simulink model "commoteur"  (Simulink 7.0)
settings: Solver=FixedStepDiscrete  StartTime=0.0  StopTime=300  FixedStep=0.0001  RelTol=1e-3
libraries: dsPICdrivers x12, simulink x5, xpcutilitieslib x2
settings Model: Creator=eleve  LastModifiedBy=eleve
settings OptimizationCC: OptimizeModelRefInitCode=on  LifeSpan=1
settings HardwareCC: ProdBitPerInt=16  ProdEndianess=LittleEndian  ProdWordSize=16  ProdHWDeviceType=16-bit Generic  TargetHWDeviceType=32-bit Generic
settings RTWCC: SystemTargetFile=dspic.tlc  TemplateMakefile=dspic_pic30_gcc.tmf  PostCodeGenCommand=dsPIC_Compile()  Description=Embedded Target for Microchip dsPIC (real-time)  ProcessScript=dspic_make_rtw_hook
settings CodeAppCC: IgnoreCustomStorageClasses=off
settings STFCustomTargetCC: GenFloatMathFcnCalls=ANSI_C  ModelReferenceCompliant=off  IncludeMdlTerminateFcn=off  CombineOutputUpdateFcns=on  SuppressErrorStatus=on  ERTCustomFileBanners=on  SupportContinuousTime=off  SupportNonInlinedSFcns=off  SystemTargetFile=dspic.tlc
settings ERTTargetCC: GenFloatMathFcnCalls=ANSI_C  ModelReferenceCompliant=off  CompOptLevelCompliant=off  IncludeMdlTerminateFcn=off  SuppressErrorStatus=on  ModelStepFunctionPrototypeControlCompliant=off  InlinedParameterPlacement=NonHierarchical  ERTSrcFileBannerTemplate=dsPIC_code_template.cgt  ERTHdrFileBannerTemplate=dsPIC_code_template.cgt  ERTDataSrcFileTemplate=dsPIC_code_template.cgt  ERTDataHdrFileTemplate=dsPIC_code_template.cgt  ERTCustomFileTemplate=dsPIC_main.tlc
settings CustomProperty: DataType=string  Value=C:\PROGRA~1\MATLAB\R2007b\bin\win32\gmake

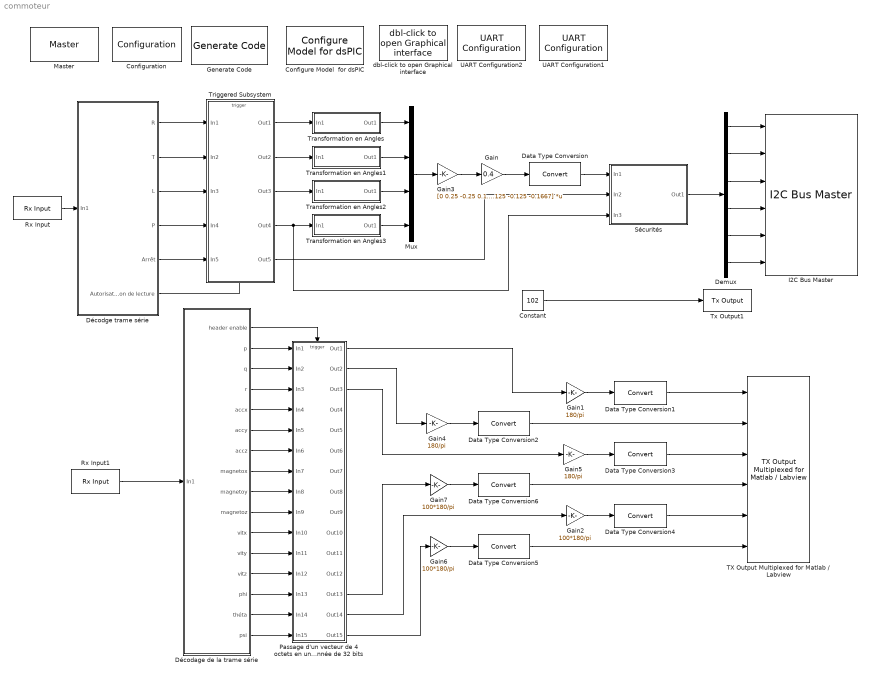
== system commoteur ==
  Configuration : dsPICdrivers/Configuration  SystemSampleTime=-1  double64=off
  Configure Model  for dsPIC : dsPICdrivers/Simulink Configuration/Configure Model  for dsPIC
  Constant : Constant  Value=102  OutDataTypeMode=uint8  OutDataType=sfix(16)  OutScaling=2^0  SampleTime=0.01
  Data Type Conversion : DataTypeConversion  OutDataTypeMode=uint8  OutDataType=sfix(16)  OutScaling=2^0
  Data Type Conversion{1..6} (6 alike) : DataTypeConversion  OutDataTypeMode=uint16  OutDataType=sfix(16)  OutScaling=2^0
  Demux : Demux  Outputs=6
  Décodage de la trame série : Subsystem  TreatAsAtomicUnit=on
  Décodge trame série : Subsystem
  Gain : Gain  Gain=0.4  ParameterDataType=sfix(16)  ParameterScaling=2^0  OutDataTypeMode=single  OutDataType=sfix(16)  OutScaling=2^0
  Gain1 : Gain  Gain=180/pi  ParameterDataType=sfix(16)  ParameterScaling=2^0  OutDataType=sfix(16)  OutScaling=2^0
  Gain2 : Gain  Gain=100*180/pi  ParameterDataType=sfix(16)  ParameterScaling=2^0  OutDataType=sfix(16)  OutScaling=2^0
  Gain3 : Gain  Gain=[0 0.25 -0.25 0.1667; 0.25 -0.125 -0.125 -0.1667; -0.25 -0.125 -0.125 0.1667; 0 0.25 -0.25 -0.1667; 0.25 -0.125 -0.125 0.1667; -0.25 -0.125 -0.125 -0.1667]  Multiplication=Matrix(K*u)  ParameterDataType=sfix(16)  ParameterScaling=2^0  OutDataTypeMode=single  OutDataType=sfix(16)  OutScaling=2^0
  Gain4 : Gain  Gain=180/pi  ParameterDataType=sfix(16)  ParameterScaling=2^0  OutDataType=sfix(16)  OutScaling=2^0
  Gain5 : Gain  Gain=180/pi  ParameterDataType=sfix(16)  ParameterScaling=2^0  OutDataType=sfix(16)  OutScaling=2^0
  Gain6 : Gain  Gain=100*180/pi  ParameterDataType=sfix(16)  ParameterScaling=2^0  OutDataType=sfix(16)  OutScaling=2^0
  Gain7 : Gain  Gain=100*180/pi  ParameterDataType=sfix(16)  ParameterScaling=2^0  OutDataType=sfix(16)  OutScaling=2^0
  Generate Code : dsPICdrivers/Simulink Configuration/Generate Code
  I2C Bus Master : dsPICdrivers/BUS I2C/I2C Bus Master  Tag=dsPIC_I2C_Master  NumI2C=1  Sequence='S A82 W P S A84 W P S A86 W P S A88 W P S A90 W P S A92 W P'  InitializeOnceOnly=When PIC is initialized (only once)  Enable=off  WaitAfterEnable=1  Disable=off  AdressNbrBits=7 bits  I2CBusFreq=50  SlewRate=off  SMBUSThreshold=off  OutputErrorFlag=off  SampleTime=-1  OrderingInOutPopup=None  Info=Fscl = 401.0025 KHz
  Master : dsPICdrivers/Master  Tag=dsPIC_MASTER  Priority=1  TimeStepType=Timer1  picType=30f4013  fcy=32e6  Quartz_33f=5e6  PLLActive_33f=off  fcyDesired_33f=0  tmr1="[1  3199  0]"  tmr1Info="Time Step : 0.0001  ;   Error : 0%  PR1=3199"  tmr2345="[0  0  0  0]"  tmr2345cfg=[-1 -1 -1 -1]  IOautoConf=on  typePort="[ 0   0   0   0   0   0   0   0   0   0   0   0   0   0   0   0  10   0   0   0   0   0   0   0   0   0   0   0   0   0   0   0   0   0   0   0   0   0   0   0   0   0   0   0   0   5   4   0   0   0   0   0   0   0   0   0   0   0   0   0   0   0   0   0   0   0   0   0   0   0   0   0   0   0   0   0   0   0   0   0   0   0  20  20   4   5   0   0   0   0   0   0   0   0   0   0   0   0   0   0   0   0   0   0   0   0   0   0   0   0   0   0 ]"  TRIS="[ 65535  65534  65535  65535  65535  65535  65535 ]"  ADPCFG=1  MasterBusyPort=None  MasterOverloadPort=B0  FOSC=XT_PLL16  ClockSwitchMonitor=Both disabled  TempProtection_33f=TEMP_ON  FPBOR=PBOR_OFF  PWRT=PWRT_OFF  MCLR=MCLR_DIS  PowerSave=off  OverrideFcy=off  NewFcy=1e6  PR2345="[65535  65535  65535  65535]"
  Mux : Mux
  Passage d'un vecteur de 4 octets en une donnée de 32 bits : Subsystem  TreatAsAtomicUnit=on
  Rx Input : dsPICdrivers/Serial PORT/Rx Input  Tag=dsPIC_RX  Priority=5  UART=2  SampleTime=0.0001  BlockingFctChk=off  OutputDefault=0  IsPresentFlagChk=off
  Rx Input1 : dsPICdrivers/Serial PORT/Rx Input  Tag=dsPIC_RX  Priority=5  UART=1  SampleTime=1e-4  BlockingFctChk=off  OutputDefault=0  IsPresentFlagChk=off
  Sécurités : Subsystem
  TX Output Multiplexed for Matlab / Labview : dsPICdrivers/Serial PORT/TX Output Multiplexed for Matlab // Labview  Tag=dsPIC_TX_Multiplexed  Priority=5  UART=2  CleverSpreadingChk=on  CleverSpreading=1  CHANNEL=[0 1 2 3 4 5]  CHANNELBLOCKED=[]  CHANNELBLOCKED_BITEWISE=0  Status=OK
  Transformation en Angles : Subsystem
  Transformation en Angles1 : Subsystem
  Transformation en Angles2 : Subsystem
  Transformation en Angles3 : Subsystem
  Triggered Subsystem : Subsystem  TreatAsAtomicUnit=on
  Tx Output1 : dsPICdrivers/Serial PORT/Tx Output  Tag=dsPIC_TX  Priority=5  UART=1  OrderingInOutPopup=None
  UART Configuration1 : dsPICdrivers/Serial PORT/UART Configuration  Tag=dsPIC_config_UART  Priority=2  UART=1  proposed_BAUD=115200  ALT_TX_RX=on  InterruptTxWhen=When Transmit Buffer is empty  TXInterruptPri=7  TxBufferSize=4  TXEN=on  InterruptRxWhen=When Receive Buffer is full (contain 4 characters)  RXInterruptPri=6  RxBufferSize=64  BAUD=115200  UxBRG=16  Info="UxBRG = 16   ||  Real Baud : 117647   ||  % error : 2.1242  ||  max 1.1765 Bytes / Step"  RealBaud=0
  UART Configuration2 : dsPICdrivers/Serial PORT/UART Configuration  Tag=dsPIC_config_UART  Priority=2  UART=2  proposed_BAUD=115200  ALT_TX_RX=off  InterruptTxWhen=When Transmit Buffer is empty  TXInterruptPri=1  TxBufferSize=4  TXEN=on  InterruptRxWhen=When Receive Buffer is full (contain 4 characters)  RXInterruptPri=5  RxBufferSize=16  BAUD=115200  UxBRG=16  Info="UxBRG = 16   ||  Real Baud : 117647   ||  % error : 2.1242  ||  max 1.1765 Bytes / Step"  RealBaud=0
  dbl-click to open Graphical interface : dsPICdrivers/Serial PORT/dbl-click to open Graphical interface  SystemSampleTime=-1  Nothing=0
  wires:
  Rx Input/1 -> Décodge trame série/1(In1)
  Décodge trame série/1(R) -> Triggered Subsystem/1(In1)
  Décodge trame série/2(T) -> Triggered Subsystem/2(In2)
  Décodge trame série/3(L) -> Triggered Subsystem/3(In3)
  Décodge trame série/4(P) -> Triggered Subsystem/4(In4)
  Triggered Subsystem/1(Out1) -> Transformation en Angles/1(In1)
  Transformation en Angles/1(Out1) -> Mux/1
  Transformation en Angles3/1(Out1) -> Mux/4
  Transformation en Angles2/1(Out1) -> Mux/3
  Triggered Subsystem/2(Out2) -> Transformation en Angles1/1(In1)
  Transformation en Angles1/1(Out1) -> Mux/2
  Mux/1 -> Gain3/1
  Gain3/1 -> Gain/1
  Gain/1 -> Data Type Conversion/1
  Data Type Conversion/1 -> Sécurités/1(In1)
  Triggered Subsystem/3(Out3) -> Transformation en Angles2/1(In1)
  Triggered Subsystem/4(Out4) -> Transformation en Angles3/1(In1), Sécurités/3(In3)
  Décodge trame série/5(Arrêt) -> Triggered Subsystem/5(In5)
  Triggered Subsystem/5(Out5) -> Sécurités/2(In2)
  Demux/1 -> I2C Bus Master/1
  Demux/3 -> I2C Bus Master/3
  Demux/4 -> I2C Bus Master/4
  Demux/5 -> I2C Bus Master/5
  Demux/6 -> I2C Bus Master/6
  Demux/2 -> I2C Bus Master/2
  Sécurités/1(Out1) -> Demux/1
  ? -> ?
  Gain1/1 -> Data Type Conversion1/1
  Décodage de la trame série/2(p) -> Passage d'un vecteur de 4 octets en une donnée de 32 bits/1(In1)
  Décodage de la trame série/3(q) -> Passage d'un vecteur de 4 octets en une donnée de 32 bits/2(In2)
  Décodage de la trame série/4(r) -> Passage d'un vecteur de 4 octets en une donnée de 32 bits/3(In3)
  Décodage de la trame série/5(accx) -> Passage d'un vecteur de 4 octets en une donnée de 32 bits/4(In4)
  Décodage de la trame série/6(accy) -> Passage d'un vecteur de 4 octets en une donnée de 32 bits/5(In5)
  Décodage de la trame série/7(accz) -> Passage d'un vecteur de 4 octets en une donnée de 32 bits/6(In6)
  Décodage de la trame série/8(magnetox) -> Passage d'un vecteur de 4 octets en une donnée de 32 bits/7(In7)
  Décodage de la trame série/10(magnetoz) -> Passage d'un vecteur de 4 octets en une donnée de 32 bits/9(In9)
  Décodage de la trame série/12(vity) -> Passage d'un vecteur de 4 octets en une donnée de 32 bits/11(In11)
  Décodage de la trame série/13(vitz) -> Passage d'un vecteur de 4 octets en une donnée de 32 bits/12(In12)
  Décodage de la trame série/14(phi) -> Passage d'un vecteur de 4 octets en une donnée de 32 bits/13(In13)
  Décodage de la trame série/15(théta) -> Passage d'un vecteur de 4 octets en une donnée de 32 bits/14(In14)
  Décodage de la trame série/9(magnetoy) -> Passage d'un vecteur de 4 octets en une donnée de 32 bits/8(In8)
  Gain4/1 -> Data Type Conversion2/1
  Gain5/1 -> Data Type Conversion3/1
  Constant/1 -> Tx Output1/1
  Gain2/1 -> Data Type Conversion4/1
  Gain6/1 -> Data Type Conversion5/1
  Gain7/1 -> Data Type Conversion6/1
  Décodage de la trame série/1(header enable) -> Passage d'un vecteur de 4 octets en une donnée de 32 bits/Trigger
  Décodage de la trame série/16(psi) -> Passage d'un vecteur de 4 octets en une donnée de 32 bits/15(In15)
  Rx Input1/1 -> Décodage de la trame série/1(In1)
  Passage d'un vecteur de 4 octets en une donnée de 32 bits/1(Out1) -> Gain1/1
  Passage d'un vecteur de 4 octets en une donnée de 32 bits/2(Out2) -> Gain4/1
  Passage d'un vecteur de 4 octets en une donnée de 32 bits/3(Out3) -> Gain5/1
  Décodage de la trame série/11(vitx) -> Passage d'un vecteur de 4 octets en une donnée de 32 bits/10(In10)
  Passage d'un vecteur de 4 octets en une donnée de 32 bits/15(Out15) -> Gain6/1
  Passage d'un vecteur de 4 octets en une donnée de 32 bits/13(Out13) -> Gain7/1
  Data Type Conversion1/1 -> TX Output Multiplexed for Matlab / Labview/1
  Data Type Conversion2/1 -> TX Output Multiplexed for Matlab / Labview/2
  Data Type Conversion3/1 -> TX Output Multiplexed for Matlab / Labview/3
  Data Type Conversion6/1 -> TX Output Multiplexed for Matlab / Labview/4
  Data Type Conversion4/1 -> TX Output Multiplexed for Matlab / Labview/5
  Data Type Conversion5/1 -> TX Output Multiplexed for Matlab / Labview/6
  Passage d'un vecteur de 4 octets en une donnée de 32 bits/14(Out14) -> Gain2/1
  Décodge trame série/6(Autorisation de lecture) -> Triggered Subsystem/Trigger

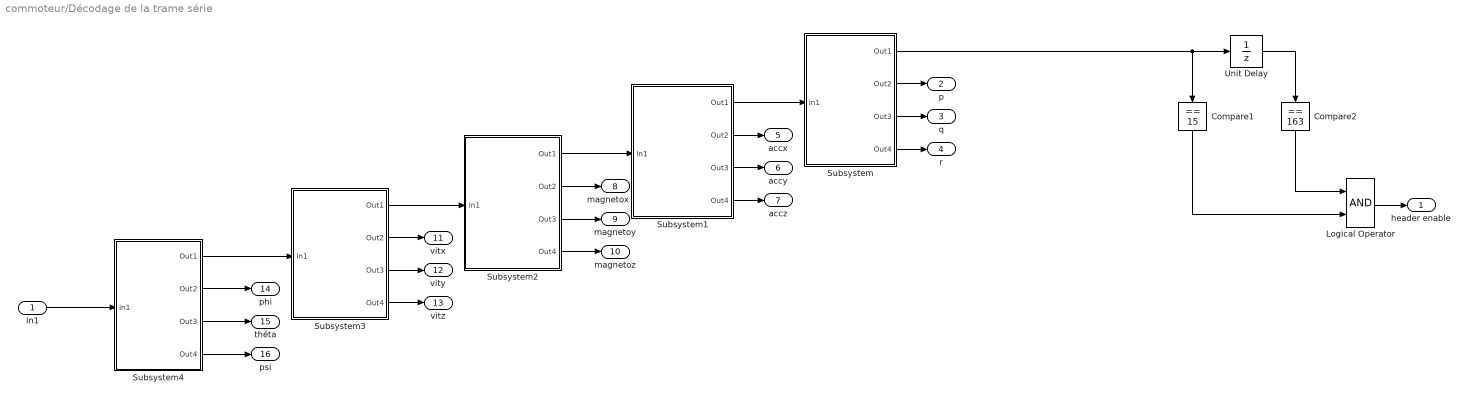
== system commoteur/Décodage de la trame série ==
  In1 : Inport  OutDataType=sfix(16)  OutScaling=2^0
  Compare1 : simulink/Logic and Bit Operations/Compare To Constant  Orientation=down  SystemSampleTime=-1  relop===  const=15  LogicOutDataTypeMode=boolean  ZeroCross=off
  Compare2 : simulink/Logic and Bit Operations/Compare To Constant  Orientation=down  SystemSampleTime=-1  relop===  const=163  LogicOutDataTypeMode=boolean  ZeroCross=off
  Logical Operator : Logic  AllPortsSameDT=off  OutDataTypeMode=boolean
  Subsystem : Subsystem
  Subsystem1 : Subsystem
  Subsystem2 : Subsystem
  Subsystem3 : Subsystem
  Subsystem4 : Subsystem
  Unit Delay : UnitDelay  SampleTime=-1
  header enable : Outport  OutDataType=sfix(16)  OutScaling=2^0
  p : Outport  Port=2  OutDataType=sfix(16)  OutScaling=2^0
  q : Outport  Port=3  OutDataType=sfix(16)  OutScaling=2^0
  r : Outport  Port=4  OutDataType=sfix(16)  OutScaling=2^0
  accx : Outport  Port=5  OutDataType=sfix(16)  OutScaling=2^0
  accy : Outport  Port=6  OutDataType=sfix(16)  OutScaling=2^0
  accz : Outport  Port=7  OutDataType=sfix(16)  OutScaling=2^0
  magnetox : Outport  Port=8  OutDataType=sfix(16)  OutScaling=2^0
  magnetoy : Outport  Port=9  OutDataType=sfix(16)  OutScaling=2^0
  magnetoz : Outport  Port=10  OutDataType=sfix(16)  OutScaling=2^0
  vitx : Outport  Port=11  OutDataType=sfix(16)  OutScaling=2^0
  vity : Outport  Port=12  OutDataType=sfix(16)  OutScaling=2^0
  vitz : Outport  Port=13  OutDataType=sfix(16)  OutScaling=2^0
  phi : Outport  Port=14  OutDataType=sfix(16)  OutScaling=2^0
  théta : Outport  Port=15  OutDataType=sfix(16)  OutScaling=2^0
  psi : Outport  Port=16  OutDataType=sfix(16)  OutScaling=2^0
  wires:
  Unit Delay/1 -> Compare2/1
  Logical Operator/1 -> header enable/1
  Compare2/1 -> Logical Operator/1
  Compare1/1 -> Logical Operator/2
  Subsystem/2(Out2) -> p/1
  Subsystem/3(Out3) -> q/1
  Subsystem/4(Out4) -> r/1
  Subsystem/1(Out1) -> Unit Delay/1, Compare1/1
  Subsystem1/1(Out1) -> Subsystem/1(In1)
  Subsystem2/1(Out1) -> Subsystem1/1(In1)
  Subsystem3/1(Out1) -> Subsystem2/1(In1)
  Subsystem4/1(Out1) -> Subsystem3/1(In1)
  Subsystem1/2(Out2) -> accx/1
  Subsystem1/3(Out3) -> accy/1
  Subsystem1/4(Out4) -> accz/1
  Subsystem2/2(Out2) -> magnetox/1
  Subsystem2/3(Out3) -> magnetoy/1
  Subsystem2/4(Out4) -> magnetoz/1
  Subsystem3/2(Out2) -> vitx/1
  Subsystem3/3(Out3) -> vity/1
  Subsystem3/4(Out4) -> vitz/1
  Subsystem4/2(Out2) -> phi/1
  Subsystem4/3(Out3) -> théta/1
  Subsystem4/4(Out4) -> psi/1
  In1/1 -> Subsystem4/1(In1)

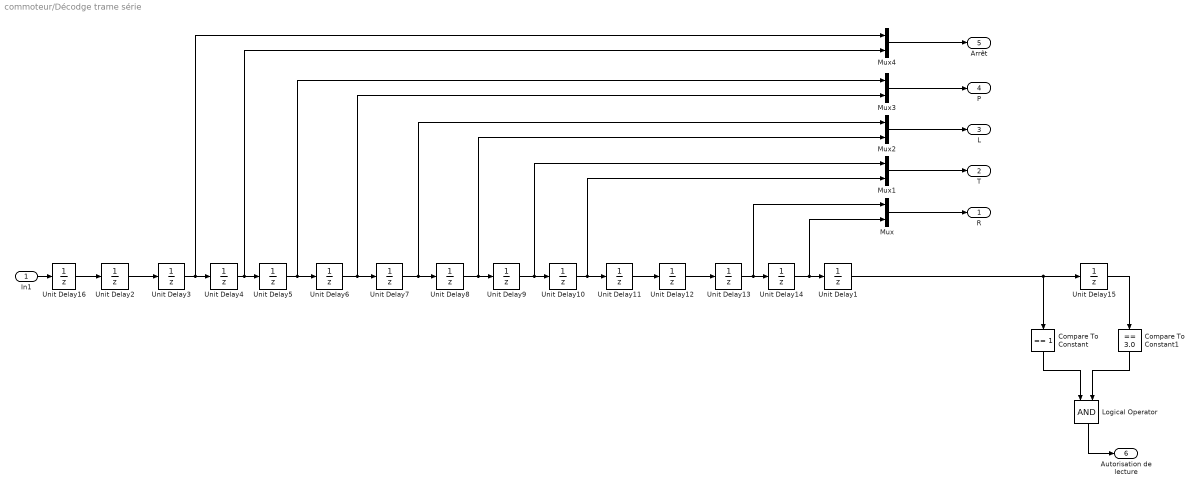
== system commoteur/Décodge trame série ==
  In1 : Inport  OutDataType=sfix(16)  OutScaling=2^0
  Compare To Constant : simulink/Logic and Bit Operations/Compare To Constant  Orientation=down  SystemSampleTime=-1  relop===  const=1  LogicOutDataTypeMode=uint8  ZeroCross=off
  Compare To Constant1 : simulink/Logic and Bit Operations/Compare To Constant  Orientation=down  SystemSampleTime=-1  relop===  const=3.0  LogicOutDataTypeMode=uint8  ZeroCross=off
  Logical Operator : Logic  Orientation=down  AllPortsSameDT=off  OutDataTypeMode=boolean
  Mux{,1..4} (5 alike) : Mux  Inputs=2
  Unit Delay{1..16} (16 alike) : UnitDelay  SampleTime=-1
  R : Outport  OutDataType=sfix(16)  OutScaling=2^0
  T : Outport  Port=2  OutDataType=sfix(16)  OutScaling=2^0
  L : Outport  Port=3  OutDataType=sfix(16)  OutScaling=2^0
  P : Outport  Port=4  OutDataType=sfix(16)  OutScaling=2^0
  Arrêt : Outport  Port=5  OutDataType=sfix(16)  OutScaling=2^0
  Autorisation de lecture : Outport  Port=6  OutDataType=sfix(16)  OutScaling=2^0
  wires:
  Unit Delay2/1 -> Unit Delay3/1
  Unit Delay3/1 -> Unit Delay4/1, Mux4/1
  Unit Delay4/1 -> Unit Delay5/1, Mux4/2
  Unit Delay6/1 -> Unit Delay7/1, Mux3/2
  Unit Delay7/1 -> Unit Delay8/1, Mux2/1
  Unit Delay8/1 -> Unit Delay9/1, Mux2/2
  Unit Delay9/1 -> Unit Delay10/1, Mux1/1
  Unit Delay10/1 -> Unit Delay11/1, Mux1/2
  Unit Delay11/1 -> Unit Delay12/1
  Unit Delay12/1 -> Unit Delay13/1
  Unit Delay13/1 -> Unit Delay14/1, Mux/1
  Unit Delay14/1 -> Unit Delay1/1, Mux/2
  Unit Delay15/1 -> Compare To Constant1/1
  Compare To Constant/1 -> Logical Operator/1
  Compare To Constant1/1 -> Logical Operator/2
  Unit Delay5/1 -> Unit Delay6/1, Mux3/1
  In1/1 -> Unit Delay16/1
  Logical Operator/1 -> Autorisation de lecture/1
  Unit Delay16/1 -> Unit Delay2/1
  Mux/1 -> R/1
  Unit Delay1/1 -> Unit Delay15/1, Compare To Constant/1
  Mux1/1 -> T/1
  Mux2/1 -> L/1
  Mux3/1 -> P/1
  Mux4/1 -> Arrêt/1

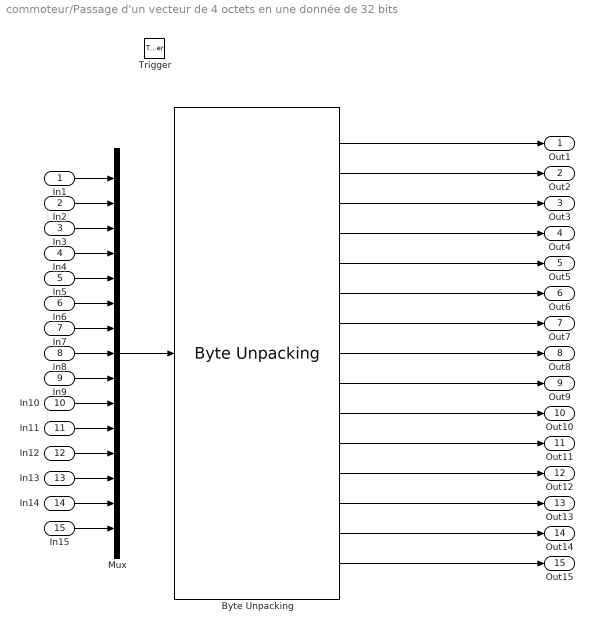
== system commoteur/Passage d'un vecteur de 4 octets en une donnée de 32 bits ==
  In1 : Inport  OutDataType=sfix(16)  OutScaling=2^0
  In2 : Inport  Port=2  OutDataType=sfix(16)  OutScaling=2^0
  In3 : Inport  Port=3  OutDataType=sfix(16)  OutScaling=2^0
  In4 : Inport  Port=4  OutDataType=sfix(16)  OutScaling=2^0
  In5 : Inport  Port=5  OutDataType=sfix(16)  OutScaling=2^0
  In6 : Inport  Port=6  OutDataType=sfix(16)  OutScaling=2^0
  In7 : Inport  Port=7  OutDataType=sfix(16)  OutScaling=2^0
  In8 : Inport  Port=8  OutDataType=sfix(16)  OutScaling=2^0
  In9 : Inport  Port=9  OutDataType=sfix(16)  OutScaling=2^0
  In10 : Inport  Port=10  OutDataType=sfix(16)  OutScaling=2^0
  In11 : Inport  Port=11  OutDataType=sfix(16)  OutScaling=2^0
  In12 : Inport  Port=12  OutDataType=sfix(16)  OutScaling=2^0
  In13 : Inport  Port=13  OutDataType=sfix(16)  OutScaling=2^0
  In14 : Inport  Port=14  OutDataType=sfix(16)  OutScaling=2^0
  In15 : Inport  Port=15  OutDataType=sfix(16)  OutScaling=2^0
  Trigger : TriggerPort
  "Byte Unpacking " : xpcutilitieslib/Byte Unpacking   MaskUnpackedDataTypes="{'single','single' ,'single' ,'single' ,'single' ,'single' ,'single' ,'single' ,'single' ,'single' ,'single' ,'single' ,'single','single' ,'single'  }"  MaskUnpackedDataSizes={1,1,1,1,1,1,1,1,1,1,1,1,1,1,1}  MaskAlignment=1
  Mux : Mux  Inputs=15
  Out1 : Outport  OutDataType=sfix(16)  OutScaling=2^0
  Out2 : Outport  Port=2  OutDataType=sfix(16)  OutScaling=2^0
  Out3 : Outport  Port=3  OutDataType=sfix(16)  OutScaling=2^0
  Out4 : Outport  Port=4  OutDataType=sfix(16)  OutScaling=2^0
  Out5 : Outport  Port=5  OutDataType=sfix(16)  OutScaling=2^0
  Out6 : Outport  Port=6  OutDataType=sfix(16)  OutScaling=2^0
  Out7 : Outport  Port=7  OutDataType=sfix(16)  OutScaling=2^0
  Out8 : Outport  Port=8  OutDataType=sfix(16)  OutScaling=2^0
  Out9 : Outport  Port=9  OutDataType=sfix(16)  OutScaling=2^0
  Out10 : Outport  Port=10  OutDataType=sfix(16)  OutScaling=2^0
  Out11 : Outport  Port=11  OutDataType=sfix(16)  OutScaling=2^0
  Out12 : Outport  Port=12  OutDataType=sfix(16)  OutScaling=2^0
  Out13 : Outport  Port=13  OutDataType=sfix(16)  OutScaling=2^0
  Out14 : Outport  Port=14  OutDataType=sfix(16)  OutScaling=2^0
  Out15 : Outport  Port=15  OutDataType=sfix(16)  OutScaling=2^0
  wires:
  "Byte Unpacking "/1 -> Out1/1
  "Byte Unpacking "/2 -> Out2/1
  "Byte Unpacking "/4 -> Out4/1
  "Byte Unpacking "/5 -> Out5/1
  "Byte Unpacking "/6 -> Out6/1
  "Byte Unpacking "/3 -> Out3/1
  Mux/1 -> "Byte Unpacking "/1
  "Byte Unpacking "/7 -> Out7/1
  "Byte Unpacking "/8 -> Out8/1
  "Byte Unpacking "/9 -> Out9/1
  "Byte Unpacking "/10 -> Out10/1
  "Byte Unpacking "/11 -> Out11/1
  "Byte Unpacking "/12 -> Out12/1
  "Byte Unpacking "/13 -> Out13/1
  "Byte Unpacking "/14 -> Out14/1
  "Byte Unpacking "/15 -> Out15/1
  In1/1 -> Mux/1
  In2/1 -> Mux/2
  In3/1 -> Mux/3
  In4/1 -> Mux/4
  In5/1 -> Mux/5
  In6/1 -> Mux/6
  In7/1 -> Mux/7
  In8/1 -> Mux/8
  In9/1 -> Mux/9
  In10/1 -> Mux/10
  In11/1 -> Mux/11
  In12/1 -> Mux/12
  In13/1 -> Mux/13
  In14/1 -> Mux/14
  In15/1 -> Mux/15

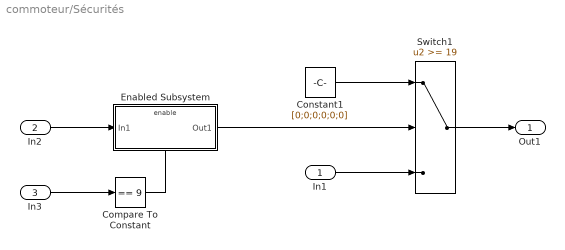
== system commoteur/Sécurités ==
  In1 : Inport
  In2 : Inport  Port=2
  In3 : Inport  Port=3  OutDataType=sfix(16)  OutScaling=2^0
  Compare To Constant : simulink/Logic and Bit Operations/Compare To Constant  SystemSampleTime=-1  relop===  const=9  LogicOutDataTypeMode=uint8  ZeroCross=off
  Constant1 : Constant  Value=[0;0;0;0;0;0]  OutDataTypeMode=uint8  OutDataType=sfix(16)  OutScaling=2^0
  Enabled Subsystem : Subsystem  TreatAsAtomicUnit=on
  Switch1 : Switch  Threshold=19  OutDataType=sfix(16)  OutScaling=2^0
  Out1 : Outport
  wires:
  Constant1/1 -> Switch1/1
  Switch1/1 -> Out1/1
  In3/1 -> Compare To Constant/1
  In2/1 -> Enabled Subsystem/1(In1)
  Enabled Subsystem/1(Out1) -> Switch1/2
  Compare To Constant/1 -> Enabled Subsystem/Enable
  In1/1 -> Switch1/3

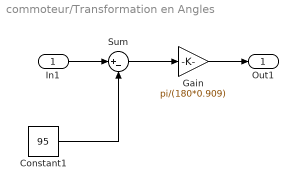
== system commoteur/Transformation en Angles ==
  In1 : Inport
  Constant1 : Constant  Value=95  OutDataTypeMode=single  OutDataType=sfix(16)  OutScaling=2^0
  Gain : Gain  Gain=pi/(180*0.909)  ParameterDataType=sfix(16)  ParameterScaling=2^0  OutDataTypeMode=single  OutDataType=sfix(16)  OutScaling=2^0
  Sum : Sum  Inputs=|+-  OutDataTypeMode=single  OutDataType=sfix(16)  OutScaling=2^0
  Out1 : Outport
  wires:
  Constant1/1 -> Sum/2
  Sum/1 -> Gain/1
  In1/1 -> Sum/1
  Gain/1 -> Out1/1

== system commoteur/Transformation en Angles1 ==
  In1 : Inport
  Constant1 : Constant  Value=159  OutDataTypeMode=single  OutDataType=sfix(16)  OutScaling=2^0
  Gain : Gain  Gain=pi/(0.909*180)  ParameterDataType=sfix(16)  ParameterScaling=2^0  OutDataTypeMode=single  OutDataType=sfix(16)  OutScaling=2^0
  Sum : Sum  Inputs=|+-  OutDataTypeMode=single  OutDataType=sfix(16)  OutScaling=2^0
  Out1 : Outport
  wires:
  Constant1/1 -> Sum/2
  Sum/1 -> Gain/1
  In1/1 -> Sum/1
  Gain/1 -> Out1/1

== system commoteur/Transformation en Angles2 ==
  In1 : Inport
  Constant1 : Constant  Value=224  OutDataTypeMode=single  OutDataType=sfix(16)  OutScaling=2^0
  Gain : Gain  Gain=pi/(0.909*180)  ParameterDataType=sfix(16)  ParameterScaling=2^0  OutDataTypeMode=single  OutDataType=sfix(16)  OutScaling=2^0
  Sum : Sum  Inputs=|+-  OutDataTypeMode=single  OutDataType=sfix(16)  OutScaling=2^0
  Out1 : Outport
  wires:
  Constant1/1 -> Sum/2
  Sum/1 -> Gain/1
  In1/1 -> Sum/1
  Gain/1 -> Out1/1

== system commoteur/Transformation en Angles3 ==
  In1 : Inport
  Constant1 : Constant  Value=530.3352  OutDataTypeMode=single  OutDataType=sfix(16)  OutScaling=2^0
  Gain : Gain  Gain=72.2568  ParameterDataType=sfix(16)  ParameterScaling=2^0  OutDataTypeMode=single  OutDataType=sfix(16)  OutScaling=2^0
  Sum : Sum  Inputs=|+-  OutDataTypeMode=single  OutDataType=sfix(16)  OutScaling=2^0
  Out1 : Outport
  wires:
  Constant1/1 -> Sum/2
  In1/1 -> Gain/1
  Sum/1 -> Out1/1
  Gain/1 -> Sum/1

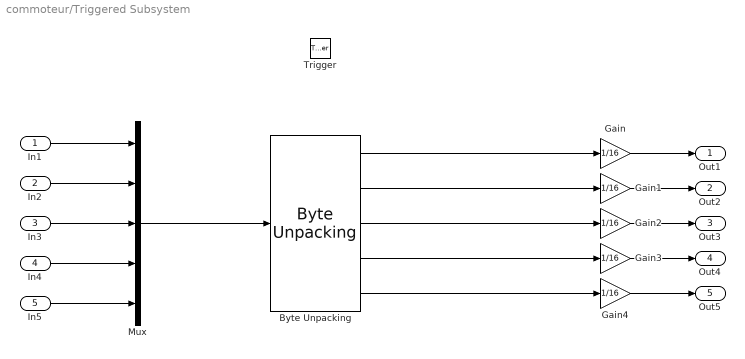
== system commoteur/Triggered Subsystem ==
  In1 : Inport  OutDataType=sfix(16)  OutScaling=2^0
  In2 : Inport  Port=2  OutDataType=sfix(16)  OutScaling=2^0
  In3 : Inport  Port=3  OutDataType=sfix(16)  OutScaling=2^0
  In4 : Inport  Port=4  OutDataType=sfix(16)  OutScaling=2^0
  In5 : Inport  Port=5  OutDataType=sfix(16)  OutScaling=2^0
  Trigger : TriggerPort
  "Byte Unpacking " : xpcutilitieslib/Byte Unpacking   MaskUnpackedDataTypes={'uint16','uint16','uint16','uint16','uint16'}  MaskUnpackedDataSizes={1,1,1,1,1}  MaskAlignment=1
  Gain{,1..4} (5 alike) : Gain  Gain=1/16  ParameterDataType=sfix(16)  ParameterScaling=2^0  OutDataTypeMode=uint8  OutDataType=sfix(16)  OutScaling=2^0
  Mux : Mux  Inputs=5
  Out1 : Outport  OutDataType=sfix(16)  OutScaling=2^0
  Out2 : Outport  Port=2  OutDataType=sfix(16)  OutScaling=2^0
  Out3 : Outport  Port=3  OutDataType=sfix(16)  OutScaling=2^0
  Out4 : Outport  Port=4  OutDataType=sfix(16)  OutScaling=2^0
  Out5 : Outport  Port=5  OutDataType=sfix(16)  OutScaling=2^0
  wires:
  Mux/1 -> "Byte Unpacking "/1
  In1/1 -> Mux/1
  In2/1 -> Mux/2
  In3/1 -> Mux/3
  In4/1 -> Mux/4
  "Byte Unpacking "/1 -> Gain/1
  "Byte Unpacking "/3 -> Gain2/1
  "Byte Unpacking "/2 -> Gain1/1
  "Byte Unpacking "/4 -> Gain3/1
  Gain/1 -> Out1/1
  Gain1/1 -> Out2/1
  Gain2/1 -> Out3/1
  Gain3/1 -> Out4/1
  Gain4/1 -> Out5/1
  "Byte Unpacking "/5 -> Gain4/1
  In5/1 -> Mux/5

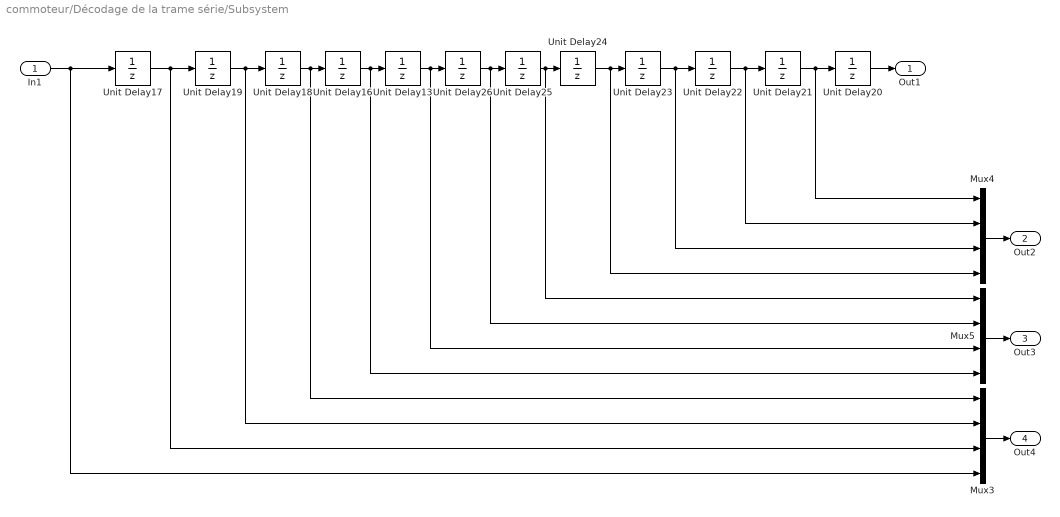
== system commoteur/Décodage de la trame série/Subsystem ==
  In1 : Inport
  Mux3 : Mux
  Mux4 : Mux
  Mux5 : Mux
  Unit Delay{13,16..26} (12 alike) : UnitDelay  SampleTime=-1
  Out1 : Outport
  Out2 : Outport  Port=2
  Out3 : Outport  Port=3
  Out4 : Outport  Port=4
  wires:
  Unit Delay21/1 -> Unit Delay20/1, Mux4/1
  Unit Delay22/1 -> Unit Delay21/1, Mux4/2
  Unit Delay23/1 -> Unit Delay22/1, Mux4/3
  Unit Delay24/1 -> Unit Delay23/1, Mux4/4
  Unit Delay25/1 -> Unit Delay24/1, Mux5/1
  Unit Delay26/1 -> Unit Delay25/1, Mux5/2
  Unit Delay13/1 -> Unit Delay26/1, Mux5/3
  Unit Delay16/1 -> Unit Delay13/1, Mux5/4
  Unit Delay19/1 -> Unit Delay18/1, Mux3/2
  Unit Delay17/1 -> Unit Delay19/1, Mux3/3
  Unit Delay18/1 -> Unit Delay16/1, Mux3/1
  In1/1 -> Unit Delay17/1, Mux3/4
  Unit Delay20/1 -> Out1/1
  Mux4/1 -> Out2/1
  Mux5/1 -> Out3/1
  Mux3/1 -> Out4/1

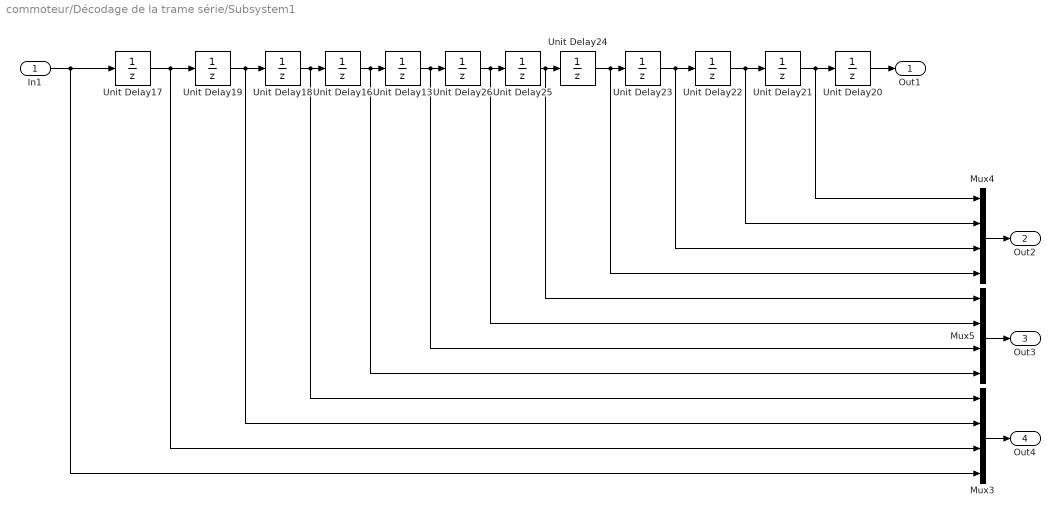
== system commoteur/Décodage de la trame série/Subsystem1 ==
  In1 : Inport
  Mux3 : Mux
  Mux4 : Mux
  Mux5 : Mux
  Unit Delay{13,16..26} (12 alike) : UnitDelay  SampleTime=-1
  Out1 : Outport
  Out2 : Outport  Port=2
  Out3 : Outport  Port=3
  Out4 : Outport  Port=4
  wires:
  Unit Delay21/1 -> Unit Delay20/1, Mux4/1
  Unit Delay22/1 -> Unit Delay21/1, Mux4/2
  Unit Delay23/1 -> Unit Delay22/1, Mux4/3
  Unit Delay24/1 -> Unit Delay23/1, Mux4/4
  Unit Delay25/1 -> Unit Delay24/1, Mux5/1
  Unit Delay26/1 -> Unit Delay25/1, Mux5/2
  Unit Delay13/1 -> Unit Delay26/1, Mux5/3
  Unit Delay16/1 -> Unit Delay13/1, Mux5/4
  Unit Delay19/1 -> Unit Delay18/1, Mux3/2
  Unit Delay17/1 -> Unit Delay19/1, Mux3/3
  Unit Delay18/1 -> Unit Delay16/1, Mux3/1
  In1/1 -> Unit Delay17/1, Mux3/4
  Unit Delay20/1 -> Out1/1
  Mux4/1 -> Out2/1
  Mux5/1 -> Out3/1
  Mux3/1 -> Out4/1

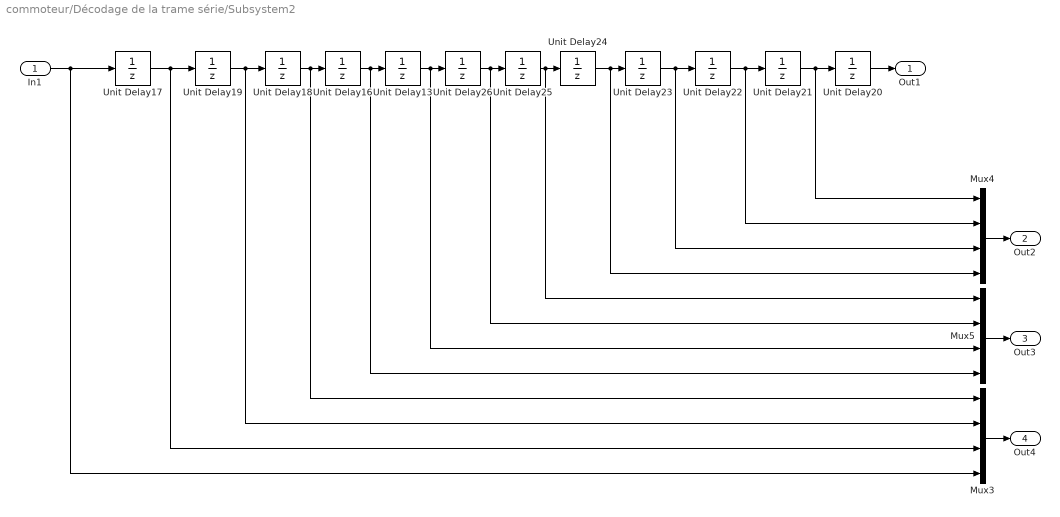
== system commoteur/Décodage de la trame série/Subsystem2 ==
  In1 : Inport
  Mux3 : Mux
  Mux4 : Mux
  Mux5 : Mux
  Unit Delay{13,16..26} (12 alike) : UnitDelay  SampleTime=-1
  Out1 : Outport
  Out2 : Outport  Port=2
  Out3 : Outport  Port=3
  Out4 : Outport  Port=4
  wires:
  Unit Delay21/1 -> Unit Delay20/1, Mux4/1
  Unit Delay22/1 -> Unit Delay21/1, Mux4/2
  Unit Delay23/1 -> Unit Delay22/1, Mux4/3
  Unit Delay24/1 -> Unit Delay23/1, Mux4/4
  Unit Delay25/1 -> Unit Delay24/1, Mux5/1
  Unit Delay26/1 -> Unit Delay25/1, Mux5/2
  Unit Delay13/1 -> Unit Delay26/1, Mux5/3
  Unit Delay16/1 -> Unit Delay13/1, Mux5/4
  Unit Delay19/1 -> Unit Delay18/1, Mux3/2
  Unit Delay17/1 -> Unit Delay19/1, Mux3/3
  Unit Delay18/1 -> Unit Delay16/1, Mux3/1
  In1/1 -> Unit Delay17/1, Mux3/4
  Unit Delay20/1 -> Out1/1
  Mux4/1 -> Out2/1
  Mux5/1 -> Out3/1
  Mux3/1 -> Out4/1

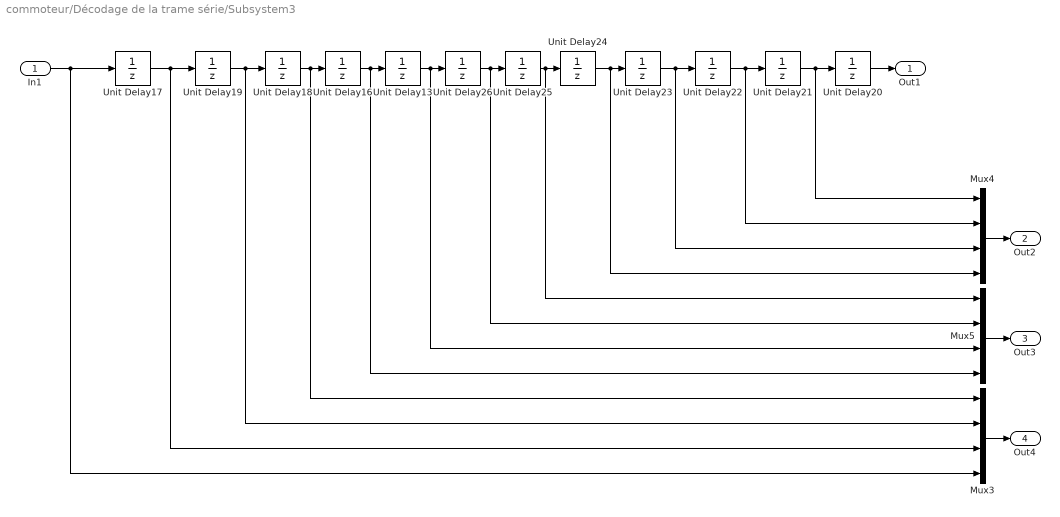
== system commoteur/Décodage de la trame série/Subsystem3 ==
  In1 : Inport
  Mux3 : Mux
  Mux4 : Mux
  Mux5 : Mux
  Unit Delay{13,16..26} (12 alike) : UnitDelay  SampleTime=-1
  Out1 : Outport
  Out2 : Outport  Port=2
  Out3 : Outport  Port=3
  Out4 : Outport  Port=4
  wires:
  Unit Delay21/1 -> Unit Delay20/1, Mux4/1
  Unit Delay22/1 -> Unit Delay21/1, Mux4/2
  Unit Delay23/1 -> Unit Delay22/1, Mux4/3
  Unit Delay24/1 -> Unit Delay23/1, Mux4/4
  Unit Delay25/1 -> Unit Delay24/1, Mux5/1
  Unit Delay26/1 -> Unit Delay25/1, Mux5/2
  Unit Delay13/1 -> Unit Delay26/1, Mux5/3
  Unit Delay16/1 -> Unit Delay13/1, Mux5/4
  Unit Delay19/1 -> Unit Delay18/1, Mux3/2
  Unit Delay17/1 -> Unit Delay19/1, Mux3/3
  Unit Delay18/1 -> Unit Delay16/1, Mux3/1
  In1/1 -> Unit Delay17/1, Mux3/4
  Unit Delay20/1 -> Out1/1
  Mux4/1 -> Out2/1
  Mux5/1 -> Out3/1
  Mux3/1 -> Out4/1

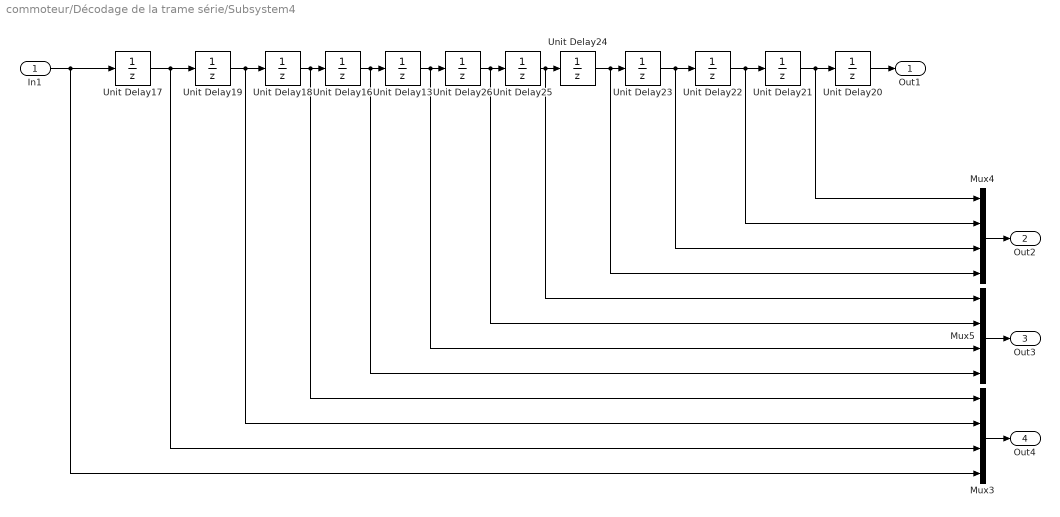
== system commoteur/Décodage de la trame série/Subsystem4 ==
  In1 : Inport
  Mux3 : Mux
  Mux4 : Mux
  Mux5 : Mux
  Unit Delay{13,16..26} (12 alike) : UnitDelay  SampleTime=-1
  Out1 : Outport
  Out2 : Outport  Port=2
  Out3 : Outport  Port=3
  Out4 : Outport  Port=4
  wires:
  Unit Delay21/1 -> Unit Delay20/1, Mux4/1
  Unit Delay22/1 -> Unit Delay21/1, Mux4/2
  Unit Delay23/1 -> Unit Delay22/1, Mux4/3
  Unit Delay24/1 -> Unit Delay23/1, Mux4/4
  Unit Delay25/1 -> Unit Delay24/1, Mux5/1
  Unit Delay26/1 -> Unit Delay25/1, Mux5/2
  Unit Delay13/1 -> Unit Delay26/1, Mux5/3
  Unit Delay16/1 -> Unit Delay13/1, Mux5/4
  Unit Delay19/1 -> Unit Delay18/1, Mux3/2
  Unit Delay17/1 -> Unit Delay19/1, Mux3/3
  Unit Delay18/1 -> Unit Delay16/1, Mux3/1
  In1/1 -> Unit Delay17/1, Mux3/4
  Unit Delay20/1 -> Out1/1
  Mux4/1 -> Out2/1
  Mux5/1 -> Out3/1
  Mux3/1 -> Out4/1

== system commoteur/Sécurités/Enabled Subsystem ==
  In1 : Inport  OutDataType=sfix(16)  OutScaling=2^0
  Enable : EnablePort
  Out1 : Outport  OutDataType=sfix(16)  OutScaling=2^0
  wires:
  In1/1 -> Out1/1
